simulink model "impl_ecu"  (R2026b)
settings: Solver=VariableStepAuto
model mask{drv=P.power.impl.mower, impl_type=1}
  mask prompts: drv "Implement drive parameters (P.power.impl.<mower|tiller>)"; impl_type "Implement type code (1 mower, 2 tiller)"
undefined symbols (not defined in the file or in its folder): DiscIntNeverNeededParam, P, Ts
libraries: simulink x14, slpidlib x1, eeGeneralControl x1
settings Model: Creator=aomar  LastModifiedBy=aomar

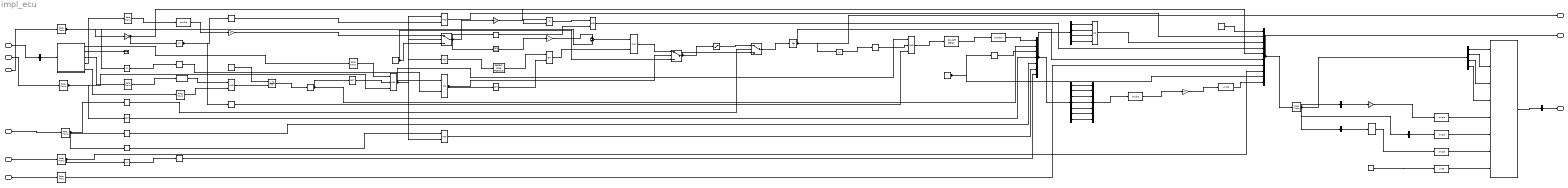
== system impl_ecu ==
  can_rx : Inport  OutDataTypeStr=Bus: Bus_Can1_McuSlow  SampleTime=Ts.can_slow
  Safety_OK : Inport  Port=2  OutDataTypeStr=boolean  SampleTime=Ts.safety
  w_motor : Inport  Port=3  OutDataTypeStr=double  SampleTime=Ts.base
  V_dc : Inport  Port=4  OutDataTypeStr=double  SampleTime=Ts.base
  I_dc : Inport  Port=5  OutDataTypeStr=double  SampleTime=Ts.base
  P_in : Inport  Port=6  OutDataTypeStr=double  SampleTime=Ts.base
  Alive_change : simulink/Logic and Bit Operations/Detect Change  vinit=0  OutDataTypeStr=boolean
  Cmd_age : DiscreteIntegrator  gainval=1  ExternalReset=level  SampleTime=Ts.impl_ctrl  LimitOutput=on  UpperSaturationLimit=P.power.impl.ecu.age_max  LowerSaturationLimit=0  ICPrevOutput=DiscIntNeverNeededParam  ICPrevScaledInput=DiscIntNeverNeededParam
  Cmd_unpack : Subsystem  ReferencedSubsystem=implcmd_can_unpack
  Disable : Logic  Operator=NOT  AllPortsSameDT=off  OutDataTypeStr=boolean
  Disable_edge : simulink/Logic and Bit Operations/Detect Rise Positive  vinit=0  OutDataTypeStr=boolean
  Drive_active : Logic  Operator=OR  AllPortsSameDT=off  OutDataTypeStr=boolean
  ECU_delay : UnitDelay  SampleTime=Ts.impl_ctrl
  Elec_BC : BusCreator  Inputs=10  OutDataTypeStr=Bus: Bus_ImplElecState  NonVirtualBus=on
      settings: InheritFromInputs=off
  Enable_eff : Logic  Inputs=3  AllPortsSameDT=off  OutDataTypeStr=boolean
  Err : Sum  Inputs=+-
  FB_BC : BusCreator  Inputs=1  OutDataTypeStr=Bus: Bus_Can1_Impl  NonVirtualBus=on
      settings: InheritFromInputs=off
  FB_I_s : DataTypeConversion  OutDataTypeStr=single  SaturateOnIntegerOverflow=off  RndMeth=Floor
  FB_I_sel : BusSelector  OutputSignals=Impl_Current_A
  FB_RT : RateTransition  OutPortSampleTime=Ts.can_slow
  FB_T_s : DataTypeConversion  OutDataTypeStr=single  SaturateOnIntegerOverflow=off  RndMeth=Floor
  FB_T_sel : BusSelector  OutputSignals=Impl_Temp_K
  FB_alive : DataTypeConversion  OutDataTypeStr=uint8  SaturateOnIntegerOverflow=off  RndMeth=Floor
  FB_alive_cnt : simulink/Sources/Counter Free-Running  NumBits=8  tsamp=Ts.can_slow
  FB_degC : Bias  Bias=-273.15  SaturateOnIntegerOverflow=off
  FB_pack : Subsystem  ReferencedSubsystem=implfb_can_pack
  FB_rpm : Gain  Gain=1/P.power.impl.rpm2rad
  FB_rpm_s : DataTypeConversion  OutDataTypeStr=single  SaturateOnIntegerOverflow=off  RndMeth=Floor
  FB_sel : BusSelector  OutputSignals=Impl_Running,Impl_Fault,Impl_Ready,Impl_Type
  FB_speed_sel : BusSelector  OutputSignals=Impl_Speed_radps
  Fault_BC : BusCreator  Inputs=7
  Fault_Code : DataTypeConversion  OutDataTypeStr=uint16  RndMeth=Nearest
  Fault_bits : Mux  Inputs=7
  Fault_bits_dbl : DataTypeConversion  OutDataTypeStr=double  SaturateOnIntegerOverflow=off  RndMeth=Floor
  Fault_bits_sel : BusSelector  OutputSignals=OC,OV,UV,OT,can_timeout,STALL,SAFETY_OFF
  Fault_reset_unused : Terminator
  Fault_weights : Gain  Gain=2.^(0:6)  Multiplication=Matrix(K*u)
  I_abs : Abs  SaturateOnIntegerOverflow=off
  Impl_Fault : Logic  Operator=OR  Inputs=4  AllPortsSameDT=off  OutDataTypeStr=boolean
  Impl_Fault_sel : BusSelector  OutputSignals=OC,OV,OT,STALL
  Inactive : Logic  Operator=NOT  AllPortsSameDT=off  OutDataTypeStr=boolean
  Moving : simulink/Logic and Bit Operations/Compare To Constant  relop=>  const=P.power.impl.ecu.run_frac*drv.w_nom*drv.ratio  OutDataTypeStr=boolean
  New_frame : Logic  AllPortsSameDT=off  OutDataTypeStr=boolean
  Not_timeout : Logic  Operator=NOT  AllPortsSameDT=off  OutDataTypeStr=boolean
  OC : simulink/Logic and Bit Operations/Compare To Constant  relop=>  const=P.power.impl.ecu.I_oc  OutDataTypeStr=boolean
  OT : simulink/Logic and Bit Operations/Compare To Constant  relop=>  const=P.power.impl.ecu.T_ot_K  OutDataTypeStr=boolean
  OV : simulink/Logic and Bit Operations/Compare To Constant  relop=>  const=P.power.impl.ecu.V_ov  OutDataTypeStr=boolean
  OV_lim : simulink/Logic and Bit Operations/Compare To Constant  relop=>  const=P.power.impl.ecu.V_ov  OutDataTypeStr=boolean
  One : Constant  SampleTime=Ts.impl_ctrl
  PI_reset : Logic  Operator=OR  AllPortsSameDT=off  OutDataTypeStr=boolean
  RT_I_dc : RateTransition  OutPortSampleTime=Ts.impl_ctrl
  RT_P_in : RateTransition  OutPortSampleTime=Ts.impl_ctrl
  RT_Safety_OK : RateTransition  OutPortSampleTime=Ts.impl_ctrl
  RT_V_dc : RateTransition  OutPortSampleTime=Ts.impl_ctrl
  RT_alive : RateTransition  OutPortSampleTime=Ts.impl_ctrl
  RT_enable : RateTransition  OutPortSampleTime=Ts.impl_ctrl
  RT_speed_rpm : RateTransition  OutPortSampleTime=Ts.impl_ctrl
  RT_valid : RateTransition  OutPortSampleTime=Ts.impl_ctrl
  RT_w_motor : RateTransition  OutPortSampleTime=Ts.impl_ctrl
  Ramp : RateLimiter  RisingSlewLimit=drv.ramp_up  FallingSlewLimit=drv.ramp_dn  SampleTimeMode=inherited
  Ratio : Gain  Gain=drv.ratio
  Ready : Logic  AllPortsSameDT=off  OutDataTypeStr=boolean
  Ready_cmp : RelationalOperator  OutDataTypeStr=boolean  RndMeth=Simplest  InputSameDT=off
  Ready_thr : Gain  Gain=P.power.impl.ecu.ready_frac
  Running : Logic  AllPortsSameDT=off  OutDataTypeStr=boolean
  Rx_sel : BusSelector  OutputSignals=impl_cmd
  SAFETY_OFF : Logic  Operator=NOT  AllPortsSameDT=off  OutDataTypeStr=boolean
  STALL : DataTypeConversion  OutDataTypeStr=boolean  RndMeth=Nearest
  Spd_dbl : DataTypeConversion  OutDataTypeStr=double  SaturateOnIntegerOverflow=off  RndMeth=Floor
  Spd_rad : Gain  Gain=P.power.impl.rpm2rad
  Speed_PI : slpidlib/PID Controller  Controller=PI  Form=Parallel  TimeDomain=Discrete-time  UseExternalTs=off  SampleTime=Ts.impl_ctrl  IntegratorMethod=Forward Euler  FilterMethod=Forward Euler  ControllerParametersSource=internal  P=drv.Kp  I=drv.Ki  UseKiTs=off  D=0  UseExternalDerivativeSource=off  N=100  UseFilter=on  TunerSelectOption=Transfer Function Based (PID Tuner App)  InitialConditionSource=internal  InitialConditionForIntegrator=0  InitialConditionForFilter=0  DifferentiatorICPrevScaledInput=0  ExternalReset=level  TrackingMode=off  Kt=1  LimitOutput=on  SatLimitsSource=internal  UpperSaturationLimit=drv.T_max  LowerSaturationLimit=-drv.T_brake  LinearizeAsGain=off  AntiWindupMode=clamping  Kb=1  LimitIntegrator=off  UpperIntegratorSaturationLimit=inf  LowerIntegratorSaturationLimit=-inf  POutMin=[]  POutMax=[]  IOutMin=[]  IOutMax=[]  DOutMin=[]  DOutMax=[]  NOutMin=[]  NOutMax=[]  SumOutMin=[]  SumOutMax=[]  SaturationOutMin=[]  SaturationOutMax=[]  PParamMin=[]  PParamMax=[]  IParamMin=[]  IParamMax=[]  DParamMin=[]  DParamMax=[]  NParamMin=[]  NParamMax=[]  KbParamMin=[]  KbParamMax=[]  KtParamMin=[]  KtParamMax=[]  KbOutMin=[]  KbOutMax=[]  KtOutMin=[]  KtOutMax=[]  IntegratorOutMin=[]  IntegratorOutMax=[]  FilterOutMin=[]  FilterOutMax=[]  SumI1OutMin=[]  SumI1OutMax=[]  SumI2OutMin=[]  SumI2OutMax=[]  SumI3OutMin=[]  SumI3OutMax=[]  SumI4OutMin=[]  SumI4OutMax=[]  SumDOutMin=[]  SumDOutMax=[]  DifferentiatorOutMin=[]  DifferentiatorOutMax=[]  FilterDiffOutCoefMin=[]  FilterDiffOutCoefMax=[]  ReciprocalOutMin=[]  ReciprocalOutMax=[]  SumDenOutMin=[]  SumDenOutMax=[]  SumNumOutMin=[]  SumNumOutMax=[]  DivideOutMin=[]  DivideOutMax=[]  UdiffTsProdOutMin=[]  UdiffTsProdOutMax=[]  NTsProdOutMin=[]  NTsProdOutMax=[]  UintegralTsProdOutMin=[]  UintegralTsProdOutMax=[]  UngainTsProdOutMin=[]  UngainTsProdOutMax=[]  ClampingZeroOutDataTypeStr=Inherit: Inherit via back propagation  ClampingZeroOutMin=[]  ClampingZeroOutMax=[]  FilterDenConstantOutDataTypeStr=Inherit: Inherit via back propagation  FilterDenConstantOutMin=[]  FilterDenConstantOutMax=[]  PCopyOutDataTypeStr=Inherit: Inherit via back propagation  PCopyOutMin=[]  PCopyOutMax=[]  NCopyOutDataTypeStr=Inherit: Inherit via back propagation  NCopyOutMin=[]  NCopyOutMax=[]  IntegratorContinuousStateAttributes=''  IntegratorStateMustResolveToSignalObject=off  IntegratorRTWStateStorageClass=Auto  FilterContinuousStateAttributes=''  FilterStateMustResolveToSignalObject=off  FilterRTWStateStorageClass=Auto  ParallelPVariant=InternalParameters  IdealPVariant=Disabled  IVariant=InternalParameters  DVariant=Disabled  IntegratorVariant=Discrete  SatVariant=Enabled  AWVariant=DiscClampingParallel  PCopyVariant=Disabled  TRVariant=Disabled  FdbkBlocksVariant=Forward  IdealPFdbkVariant=Disabled  SatFdbkVariant=Disabled  DerivativeFilterVariant=Disabled  NVariant=Disabled  NCopyVariant=Disabled_SignalSpec  FilterICVariant=Disabled  IntegratorICVariant=InternalICs  ExternalResetVariant=ExternalReset  TRSumVariant=Passthrough  SumFdbkVariant=Disabled  SumVariant=Sum_PI  TsampFilterVariant=InternalTs  TsampNgainVariant=Passthrough  TsampIntegralVariant=Disabled_SignalSpec  ExternalSaturationOutDataTypeStr=Inherit: Same as second input  DerivativeSourceVariant=Disabled  PreIntVariant=InternalPreInt
      settings: LibrarySourceBlock=simulink/Discrete/Discrete PID Controller
  Spinning : simulink/Logic and Bit Operations/Compare To Constant  relop=>  const=P.power.impl.ecu.run_frac*drv.w_nom  OutDataTypeStr=boolean
  Stall_cond : Logic  Inputs=3  AllPortsSameDT=off  OutDataTypeStr=boolean
  Stall_timer : eeGeneralControl/On-Off Delay  LabelModeActiveChoice=Discrete  Td_on=P.power.impl.ecu.t_stall  Td_off=0  IC=0  Ts=Ts.impl_ctrl
      settings: LibrarySourceBlock=ee_sl_lib/General Control/On-Off Delay
  T_abs : Abs  SaturateOnIntegerOverflow=off
  T_active : Switch  Criteria=u2 ~= 0  SaturateOnIntegerOverflow=off  InputSameDT=off
  T_at_lim : simulink/Logic and Bit Operations/Compare To Constant  relop=>=  const=P.power.impl.ecu.stall_T_frac*drv.T_max  OutDataTypeStr=boolean
  T_motor : Constant  Value=P.power.impl.ecu.T_motor_K  SampleTime=Ts.impl_ctrl
  T_motoring : Saturate  UpperLimit=inf  LowerLimit=0
  T_ovp : Switch  Criteria=u2 ~= 0  SaturateOnIntegerOverflow=off  InputSameDT=off
  Target : Switch  Criteria=u2 ~= 0  SaturateOnIntegerOverflow=off  InputSameDT=off
  Target_pos : simulink/Logic and Bit Operations/Compare To Constant  relop=>  const=0  OutDataTypeStr=boolean
  Timeout : simulink/Logic and Bit Operations/Compare To Constant  relop=>=  const=P.power.impl.ecu.t_can_timeout - 1e-9  OutDataTypeStr=boolean
  Type : Constant  Value=impl_type  OutDataTypeStr=uint8  SampleTime=Ts.impl_ctrl
  UV : Logic  AllPortsSameDT=off  OutDataTypeStr=boolean
  V_low : simulink/Logic and Bit Operations/Compare To Constant  relop=<  const=P.power.impl.ecu.V_uv  OutDataTypeStr=boolean
  W_abs : Abs  SaturateOnIntegerOverflow=off
  W_abs_ctl : Abs  SaturateOnIntegerOverflow=off
  W_low : simulink/Logic and Bit Operations/Compare To Constant  relop=<  const=P.power.impl.ecu.stall_frac*drv.w_nom  OutDataTypeStr=boolean
  W_shaft : Gain  Gain=1/drv.ratio
  Zero : Constant  Value=0  SampleTime=Ts.impl_ctrl
  T_ref : Outport  OutDataTypeStr=double
  impl_elec : Outport  Port=2  OutDataTypeStr=Bus: Bus_ImplElecState
  can_tx : Outport  Port=3  OutDataTypeStr=Bus: Bus_Can1_Impl
  wires:
  can_rx/1 -> Rx_sel/1  "can_rx"
  Safety_OK/1 -> RT_Safety_OK/1  "Safety_OK"
  w_motor/1 -> RT_w_motor/1  "w_motor"
  V_dc/1 -> RT_V_dc/1  "V_dc"
  I_dc/1 -> RT_I_dc/1  "I_dc"
  P_in/1 -> RT_P_in/1  "P_in"
  Rx_sel/1 -> Cmd_unpack/1  "<impl_cmd>"
  RT_w_motor/1 -> W_abs_ctl/1, Err/2, W_shaft/1  "w_motor_10ms"
  RT_I_dc/1 -> Elec_BC/8, I_abs/1  "Impl_Current_A"
  RT_P_in/1 -> Elec_BC/7  "Impl_Power_W"
  RT_Safety_OK/1 -> SAFETY_OFF/1, Enable_eff/3  "Safety_OK_10ms"
  RT_V_dc/1 -> OV_lim/1, V_low/1, OV/1  "V_dc_10ms"
  Cmd_unpack/1 -> RT_enable/1  "enable"
  Cmd_unpack/2 -> Fault_reset_unused/1  "fault_reset"
  Cmd_unpack/3 -> RT_alive/1  "alive"
  Cmd_unpack/4 -> RT_speed_rpm/1  "speed_rpm"
  Cmd_unpack/5 -> RT_valid/1  "valid"
  W_shaft/1 -> Ready_cmp/1, Elec_BC/5, W_abs/1  "Impl_Speed_radps"
  W_abs_ctl/1 -> Moving/1  "w_motor_abs"
  OV_lim/1 -> T_ovp/2  "dc_overvoltage"
  SAFETY_OFF/1 -> Fault_BC/4  "SAFETY_OFF"
  OV/1 -> Fault_BC/5  "OV"
  V_low/1 -> UV/1  "v_low"
  I_abs/1 -> OC/1  "I_dc_abs"
  RT_speed_rpm/1 -> Spd_dbl/1  "speed_rpm_10ms"
  RT_alive/1 -> Alive_change/1  "alive_10ms"
  W_abs/1 -> W_low/1, Spinning/1  "w_shaft_abs"
  Moving/1 -> Drive_active/2  "moving"
  OC/1 -> Fault_BC/7  "OC"
  RT_valid/1 -> New_frame/2  "valid_10ms"
  Alive_change/1 -> New_frame/1  "alive_changed"
  Spd_dbl/1 -> Spd_rad/1  "speed_rpm_dbl"
  Spinning/1 -> Running/2  "spinning"
  Spd_rad/1 -> Target/1  "w_cmd"
  One/1 -> Cmd_age/1  "one"
  New_frame/1 -> Cmd_age/2  "new_frame"
  W_low/1 -> Stall_cond/3  "w_low"
  Cmd_age/1 -> Timeout/1  "cmd_age"
  Timeout/1 -> Fault_BC/2, Not_timeout/1  "can_timeout"
  Not_timeout/1 -> Enable_eff/2  "can_ok"
  RT_enable/1 -> Enable_eff/1  "enable_10ms"
  Enable_eff/1 -> Running/1, UV/2, Target/2, Stall_cond/1, Disable/1, Drive_active/1  "enable_eff"
  Zero/1 -> Target/3, T_active/3  "zero"
  Running/1 -> Elec_BC/2  "Impl_Running"
  Disable/1 -> Disable_edge/1  "disable"
  Drive_active/1 -> T_active/2, Inactive/1  "drive_active"
  UV/1 -> Fault_BC/6  "UV"
  Target/1 -> Ready_thr/1, Ramp/1, Target_pos/1  "w_target"
  Ready_thr/1 -> Ready_cmp/2  "w_ready"
  Target_pos/1 -> Ready/2  "target_pos"
  Ramp/1 -> Ratio/1  "w_ref_shaft"
  Inactive/1 -> PI_reset/2  "inactive"
  Disable_edge/1 -> PI_reset/1  "disable_edge"
  Ready_cmp/1 -> Ready/1  "at_speed"
  Ratio/1 -> Err/1  "w_ref_motor"
  PI_reset/1 -> Speed_PI/2  "pi_reset"
  Err/1 -> Speed_PI/1  "w_err"
  Ready/1 -> Elec_BC/4  "Impl_Ready"
  Speed_PI/1 -> T_active/1  "T_pi"
  T_active/1 -> T_motoring/1, T_ovp/3  "T_active"
  T_motoring/1 -> T_ovp/1  "T_motoring"
  T_ovp/1 -> ECU_delay/1  "T_cmd"
  ECU_delay/1 -> T_ref/1, Elec_BC/6, T_abs/1  "Impl_Torque_Nm"
  T_abs/1 -> T_at_lim/1  "T_ref_abs"
  T_at_lim/1 -> Stall_cond/2  "T_at_lim"
  Stall_cond/1 -> Stall_timer/1  "stall_cond"
  T_motor/1 -> OT/1, Elec_BC/9  "Impl_Temp_K"
  Stall_timer/1 -> STALL/1  "stall_timer"
  OT/1 -> Fault_BC/3  "OT"
  STALL/1 -> Fault_BC/1  "STALL"
  Fault_BC/1 -> Fault_bits_sel/1, Impl_Fault_sel/1  "fault_flags"
  Impl_Fault_sel/1 -> Impl_Fault/1  "<OC>"
  Impl_Fault_sel/2 -> Impl_Fault/2  "<OV>"
  Impl_Fault_sel/3 -> Impl_Fault/3  "<OT>"
  Impl_Fault_sel/4 -> Impl_Fault/4  "<STALL>"
  Fault_bits_sel/1 -> Fault_bits/1  "<OC>"
  Fault_bits_sel/2 -> Fault_bits/2  "<OV>"
  Fault_bits_sel/3 -> Fault_bits/3  "<UV>"
  Fault_bits_sel/4 -> Fault_bits/4  "<OT>"
  Fault_bits_sel/5 -> Fault_bits/5  "<can_timeout>"
  Fault_bits_sel/6 -> Fault_bits/6  "<STALL>"
  Fault_bits_sel/7 -> Fault_bits/7  "<SAFETY_OFF>"
  Fault_bits/1 -> Fault_bits_dbl/1  "fault_bits"
  Impl_Fault/1 -> Elec_BC/3  "Impl_Fault"
  Fault_bits_dbl/1 -> Fault_weights/1  "fault_bits_dbl"
  Fault_weights/1 -> Fault_Code/1  "fault_word"
  Type/1 -> Elec_BC/1  "Impl_Type"
  Fault_Code/1 -> Elec_BC/10  "Fault_Code"
  Elec_BC/1 -> FB_RT/1, impl_elec/1  "impl_elec"
  FB_RT/1 -> FB_sel/1, FB_I_sel/1, FB_T_sel/1, FB_speed_sel/1  "impl_elec_50ms"
  FB_speed_sel/1 -> FB_rpm/1  "<Impl_Speed_radps>"
  FB_T_sel/1 -> FB_degC/1  "<Impl_Temp_K>"
  FB_rpm/1 -> FB_rpm_s/1  "speed_rpm"
  FB_alive_cnt/1 -> FB_alive/1  "alive_count"
  FB_degC/1 -> FB_T_s/1  "temp_degC"
  FB_I_sel/1 -> FB_I_s/1  "<Impl_Current_A>"
  FB_rpm_s/1 -> FB_pack/5  "speed_rpm_s"
  FB_I_s/1 -> FB_pack/6  "current_A"
  FB_T_s/1 -> FB_pack/7  "temp_degC_s"
  FB_alive/1 -> FB_pack/8  "alive"
  FB_sel/1 -> FB_pack/1  "<Impl_Running>"
  FB_sel/2 -> FB_pack/2  "<Impl_Fault>"
  FB_sel/3 -> FB_pack/3  "<Impl_Ready>"
  FB_sel/4 -> FB_pack/4  "<Impl_Type>"
  FB_pack/1 -> FB_BC/1  "impl_fb"
  FB_BC/1 -> can_tx/1  "can_tx"
